simulink model "Lazo_sc"  (R2023a)
settings: Solver=VariableStepAuto  StartTime=0.0  StopTime=4*3600  RelTol=1e-3
values from neighbouring files (symbols this model uses):
  d0 = cfg.d    [controlador_sobrecalentador_10_comparacion.m]
  dSP = cfg.dSP    [controlador_sobrecalentador_10_comparacion.m]
  du_max = p.u_max - u_ini    [controlador_sobrecalentador_10_comparacion.m]
  du_min = p.u_min - u_ini    [controlador_sobrecalentador_10_comparacion.m]
  K_u = p.K_u    [controlador_sobrecalentador_10_comparacion.m]    (also in identificacion_paso3.m = K_kW*dQdu)
  Kc = ctrl(i).Kc    [controlador_sobrecalentador_10_comparacion.m]
  KD = ctrl(i).KD    [controlador_sobrecalentador_10_comparacion.m]
  KI = ctrl(i).KI    [controlador_sobrecalentador_10_comparacion.m]
  Nf = 1    [controlador_sobrecalentador_10_comparacion.m]
  t_d = cfg.t_d    [controlador_sobrecalentador_10_comparacion.m]
  t_sp = cfg.t_sp    [controlador_sobrecalentador_10_comparacion.m]
  tau1 = p.tau1    [controlador_sobrecalentador_10_comparacion.m]    (also in identificacion_paso3.m = max(m2.Tp1, m2.Tp2))
  tau2 = p.tau2    [controlador_sobrecalentador_10_comparacion.m]    (also in identificacion_paso3.m = min(m2.Tp1, m2.Tp2))
  theta0 = p.theta0    [controlador_sobrecalentador_10_comparacion.m]    (also in identificacion_paso3.m = m2.Td)
  Ts = cfg.Ts    [comparacion_modelo_fisico.m]    (also in controlador_sobrecalentador_10_comparacion.m; identificacion_paso1.m = 10)
  u_ini = cfg.u_ini    [controlador_sobrecalentador_10_comparacion.m]
  y_ini = x0(3)    [comparacion_modelo_fisico.m]    (also in controlador_sobrecalentador_10_comparacion.m = p.Tv0 + p.K_u*(cfg.u_ini - p.u0))
libraries: slpidlib x1
settings Model: Creator=Pablo  LastModifiedBy=Pablo

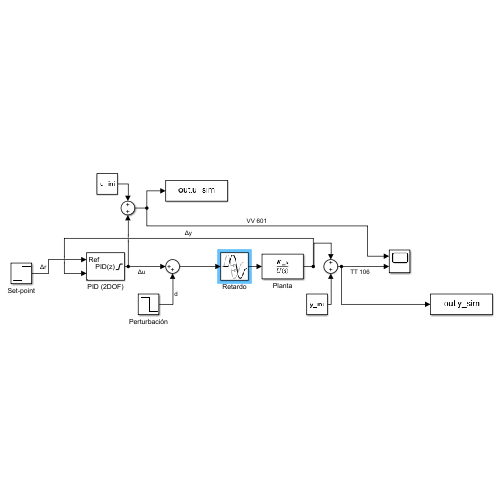
[thumbnail: Simulink's stored preview of the top-level diagram]
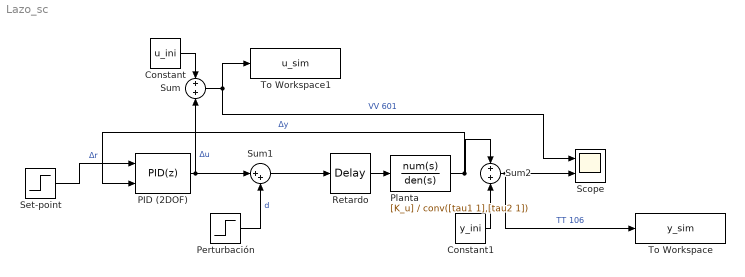
== system Lazo_sc ==
  Constant : Constant  Value=u_ini
  Constant1 : Constant  Value=y_ini
  PID (2DOF) : slpidlib/PID Controller (2DOF)  Controller=PID  Form=Parallel  TimeDomain=Discrete-time  UseExternalTs=off  SampleTime=Ts  IntegratorMethod=Forward Euler  FilterMethod=Forward Euler  ControllerParametersSource=internal  P=Kc  I=KI  UseKiTs=off  D=KD  N=Nf  UseFilter=on  b=1  c=0  TunerSelectOption=Transfer Function Based (PID Tuner App)  InitialConditionSource=internal  InitialConditionForIntegrator=0  InitialConditionForFilter=0  DifferentiatorICPrevScaledInput=0  ExternalReset=none  TrackingMode=off  Kt=1  LimitOutput=on  SatLimitsSource=internal  UpperSaturationLimit=du_max  LowerSaturationLimit=du_min  LinearizeAsGain=on  AntiWindupMode=clamping  Kb=1  LimitIntegrator=off  UpperIntegratorSaturationLimit=inf  LowerIntegratorSaturationLimit=-inf  POutMin=[]  POutMax=[]  IOutMin=[]  IOutMax=[]  DOutMin=[]  DOutMax=[]  NOutMin=[]  NOutMax=[]  bOutMin=[]  bOutMax=[]  cOutMin=[]  cOutMax=[]  SumOutMin=[]  SumOutMax=[]  SaturationOutMin=[]  SaturationOutMax=[]  PParamMin=[]  PParamMax=[]  IParamMin=[]  IParamMax=[]  DParamMin=[]  DParamMax=[]  NParamMin=[]  NParamMax=[]  bParamMin=[]  bParamMax=[]  cParamMin=[]  cParamMax=[]  KbParamMin=[]  KbParamMax=[]  KtParamMin=[]  KtParamMax=[]  KbOutMin=[]  KbOutMax=[]  KtOutMin=[]  KtOutMax=[]  IntegratorOutMin=[]  IntegratorOutMax=[]  FilterOutMin=[]  FilterOutMax=[]  SumI1OutMin=[]  SumI1OutMax=[]  SumI2OutMin=[]  SumI2OutMax=[]  SumI3OutMin=[]  SumI3OutMax=[]  SumI4OutMin=[]  SumI4OutMax=[]  SumDOutMin=[]  SumDOutMax=[]  Sum1OutMin=[]  Sum1OutMax=[]  Sum2OutMin=[]  Sum2OutMax=[]  Sum3OutMin=[]  Sum3OutMax=[]  DifferentiatorOutMin=[]  DifferentiatorOutMax=[]  FilterDiffOutCoefMin=[]  FilterDiffOutCoefMax=[]  ReciprocalOutMin=[]  ReciprocalOutMax=[]  SumDenOutMin=[]  SumDenOutMax=[]  SumNumOutMin=[]  SumNumOutMax=[]  DivideOutMin=[]  DivideOutMax=[]  UdiffTsProdOutMin=[]  UdiffTsProdOutMax=[]  NTsProdOutMin=[]  NTsProdOutMax=[]  UintegralTsProdOutMin=[]  UintegralTsProdOutMax=[]  UngainTsProdOutMin=[]  UngainTsProdOutMax=[]  ClampingZeroOutDataTypeStr=Inherit: Inherit via back propagation  ClampingZeroOutMin=[]  ClampingZeroOutMax=[]  FilterDenConstantOutDataTypeStr=Inherit: Inherit via back propagation  FilterDenConstantOutMin=[]  FilterDenConstantOutMax=[]  PCopyOutDataTypeStr=Inherit: Inherit via back propagation  PCopyOutMin=[]  PCopyOutMax=[]  NCopyOutDataTypeStr=Inherit: Inherit via back propagation  NCopyOutMin=[]  NCopyOutMax=[]  IntegratorContinuousStateAttributes=''  IntegratorStateMustResolveToSignalObject=off  IntegratorRTWStateStorageClass=Auto  FilterContinuousStateAttributes=''  FilterStateMustResolveToSignalObject=off  FilterRTWStateStorageClass=Auto  ParallelPVariant=InternalParameters  IdealPVariant=Disabled  IVariant=InternalParameters  DVariant=InternalParameters  bVariant=InternalParameters  cVariant=InternalParameters  IntegratorVariant=Discrete  SatVariant=Enabled  AWVariant=DiscClampingParallel  PCopyVariant=Disabled  TRVariant=Disabled  FdbkBlocksVariant=Forward  IdealPFdbkVariant=Disabled  SatFdbkVariant=Disabled  DerivativeFilterVariant=ForwardEulerFilter  NVariant=InternalParameters  NCopyVariant=Disabled  FilterICVariant=InternalICsFilter  IntegratorICVariant=InternalICs  ExternalResetVariant=Disabled  TRSumVariant=Passthrough  SumFdbkVariant=Disabled  SumVariant=Sum_PID  TsampFilterVariant=InternalTs  TsampNgainVariant=Passthrough  TsampIntegralVariant=Disabled_SignalSpec  ExternalSaturationOutDataTypeStr=Inherit: Same as second input
  Perturbación : Step  Time=t_d  After=d0  SampleTime=0
  Planta : TransferFcn  Numerator=[K_u]  Denominator=conv([tau1 1],[tau2 1])
  Retardo : TransportDelay  DelayTime=theta0
  Scope : Scope  NumInputPorts=2
  Set-point : Step  Time=t_sp  After=dSP  SampleTime=0
  Sum : Sum
  Sum1 : Sum  Inputs=|++
  Sum2 : Sum
  To Workspace : ToWorkspace  VariableName=y_sim  SaveFormat=Timeseries  SampleTime=Ts
  To Workspace1 : ToWorkspace  VariableName=u_sim  SaveFormat=Timeseries  SampleTime=Ts
  wires:
  Planta/1 -> PID (2DOF)/2, Sum2/1  "Δy"
  Sum2/1 -> To Workspace/1, Scope/2  "TT 106"
  Perturbación/1 -> Sum1/2  "d"
  Constant1/1 -> Sum2/2
  Retardo/1 -> Planta/1
  Set-point/1 -> PID (2DOF)/1  "Δr"
  PID (2DOF)/1 -> Sum1/1, Sum/2  "Δu"
  Sum1/1 -> Retardo/1
  Sum/1 -> Scope/1, To Workspace1/1  "VV 601"
  Constant/1 -> Sum/1
